simulink model "W09_E2_GainMargin"  (R2024b)
settings: Solver=ode45  StartTime=0.0  StopTime=t_end  MaxStep=0.02  RelTol=1e-3
PreLoadFcn:
  | % W09_E2_GainMargin 기본 파라미터 (모델을 열 때 자동 실행)
  | defs = { 'K',0.5 ; 't_end',60 ;
  |          'numG',1 ; 'denG',[1 2 1 0] };
  | for ii = 1:size(defs,1)
  |     if ~evalin('base', sprintf('exist(''%s'',''var'')', defs{ii,1}))
  |         assignin('base', defs{ii,1}, defs{ii,2});
  |     end
  | end
  | clear defs ii
values from neighbouring files (symbols this model uses):
  K = 0.5    [W09_02_pm_to_time.m]    (also in W09_03_run_simulink.m; W09_07_examples.m)
undefined symbols (not defined in the file or in its folder): denG, numG
settings Model: Creator=admin  LastModifiedBy=admin

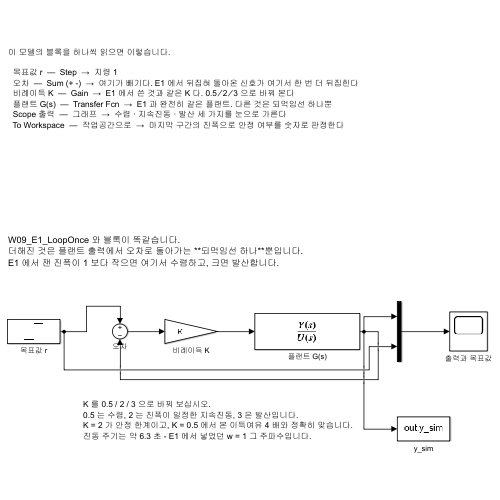
[thumbnail: Simulink's stored preview of the top-level diagram]
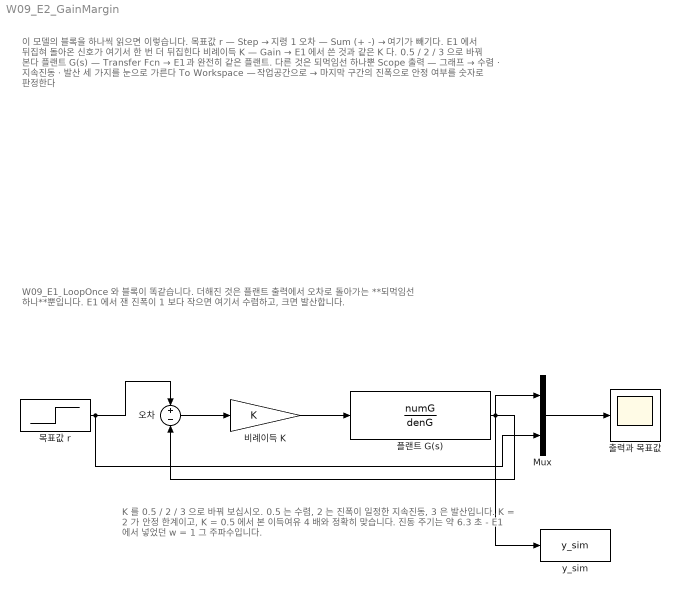
== system W09_E2_GainMargin ==
  note: W09_E1_LoopOnce 와 블록이 똑같습니다.
      | 더해진 것은 플랜트 출력에서 오차로 돌아가는 **되먹임선 하나**뿐입니다.
      | E1 에서 잰 진폭이 1 보다 작으면 여기서 수렴하고, 크면 발산합니다.
  note: K 를 0.5 / 2 / 3 으로 바꿔 보십시오.
      | 0.5 는 수렴, 2 는 진폭이 일정한 지속진동, 3 은 발산입니다.
      | K = 2 가 안정 한계이고, K = 0.5 에서 본 이득여유 4 배와 정확히 맞습니다.
      | 진동 주기는 약 6.3 초 - E1 에서 넣었던 w = 1 그 주파수입니다.
  note: 이 모델의 블록을 하나씩 읽으면 이렇습니다.
      |
      |   목표값 r  —  Step  →  지령 1
      |   오차  —  Sum (+ -)  →  여기가 빼기다. E1 에서 뒤집혀 돌아온 신호가 여기서 한 번 더 뒤집힌다
      |   비례이득 K  —  Gain  →  E1 에서 쓴 것과 같은 K 다. 0.5 ∕ 2 ∕ 3 으로 바꿔 본다
      |   플랜트 G(s)  —  Transfer Fcn  →  E1 과 완전히 같은 플랜트. 다른 것은 되먹임선 하나뿐
      |   Scope 출력  —  그래프  →  수렴 · 지속진동 · 발산 세 가지를 눈으로 가른다
      |   To Workspace  —  작업공간으로  →  마지막 구간의 진폭으로 안정 여부를 숫자로 판정한다
  Mux : Mux  Inputs=2
  y_sim : ToWorkspace  VariableName=y_sim  SaveFormat=Timeseries  SampleTime=-1
  목표값 r : Step  Time=0  SampleTime=0
  비례이득 K : Gain  Gain=K
  오차 : Sum  Inputs=+-
  출력과 목표값 : Scope
  플랜트 G(s) : TransferFcn  Numerator=numG  Denominator=denG
  wires:
  목표값 r/1 -> 오차/1, Mux/2
  오차/1 -> 비례이득 K/1
  비례이득 K/1 -> 플랜트 G(s)/1
  플랜트 G(s)/1 -> 오차/2, Mux/1, y_sim/1
  Mux/1 -> 출력과 목표값/1
